simulink model "simulink_scheme_task32"  (R2023b)
settings: Solver=ode4  StartTime=0.0  StopTime=simulationParameters.T_sim  FixedStep=simulationParameters.T_integration  RelTol=1e-3
values from neighbouring files (symbols this model uses):
  nInput = size(B,2)    [buildCondMatrices.m]    (also in main_task31.m; main_task32.m; main_task33.m)
  patientParameters = loadPatientParameter('patient#001')    [main_task32.m]    (also in main_task33.m = loadPatientParameter(patientName))
  predictedHorizon = 100    [main_task31.m]    (also in main_task32.m; main_task33.m)
  predictionData = buildCondMatrices(A,B,C,Q,R,F,f,predictedHorizon)    [main_task31.m]    (also in main_task32.m; main_task33.m)
  simulationParameters = loadSimulationParameter    [main_task31.m]    (also in main_task32.m; main_task33.m)
undefined symbols (not defined in the file or in its folder): MPCcontroller
settings Model: Creator=william  LastModifiedBy=william
settings DataIOCC: ReturnWorkspaceOutputs=off
settings ConfigComp: CovBoundaryAbsTol=1.0e-5

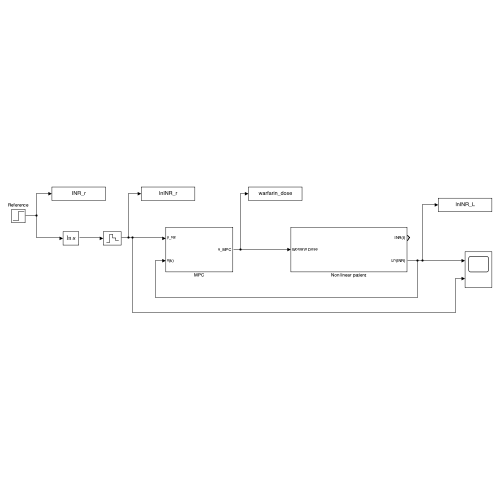
[thumbnail: Simulink's stored preview of the top-level diagram]
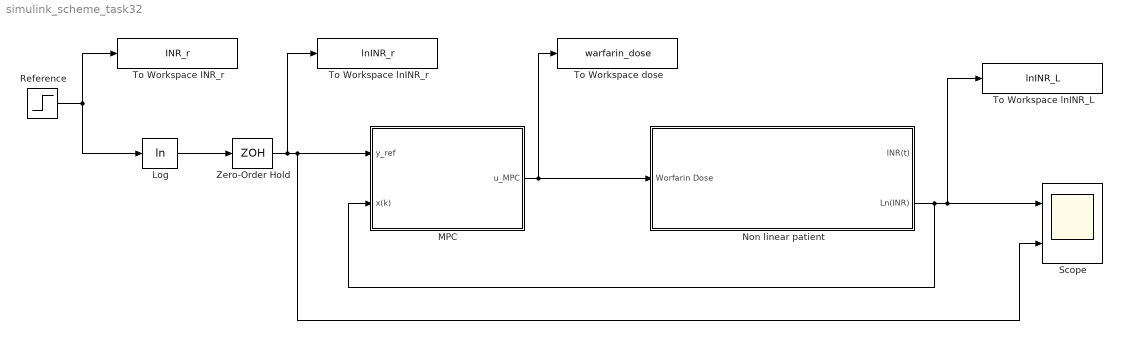
== system simulink_scheme_task32 ==
  Log : Math  Operator=log
  MPC : Subsystem
  Non linear patient : Subsystem
  Reference : Step  Time=2*24  Before=1  After=2.5  SampleTime=simulationParameters.Ts
  Scope : Scope  NumInputPorts=2
  To Workspace INR_r : ToWorkspace  VariableName=INR_r  SaveFormat=Structure With Time  SampleTime=-1
  To Workspace dose : ToWorkspace  VariableName=warfarin_dose  SaveFormat=Structure With Time  SampleTime=-1
  To Workspace lnINR_L : ToWorkspace  VariableName=lnINR_L  SaveFormat=Structure With Time  SampleTime=-1
  To Workspace lnINR_r : ToWorkspace  VariableName=lnINR_r  SaveFormat=Structure With Time  SampleTime=-1
  Zero-Order Hold : ZeroOrderHold  SampleTime=simulationParameters.Ts
  wires:
  Reference/1 -> Log/1, To Workspace INR_r/1
  Log/1 -> Zero-Order Hold/1
  Zero-Order Hold/1 -> Scope/2, MPC/1(y_ref), To Workspace lnINR_r/1
  MPC/1(u_MPC) -> Non linear patient/1(Worfarin Dose), To Workspace dose/1
  Non linear patient/2(Ln(INR)) -> To Workspace lnINR_L/1, Scope/1, MPC/2(x(k))

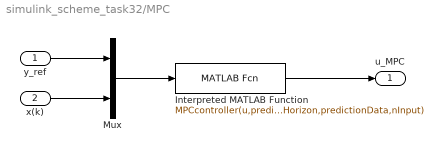
== system simulink_scheme_task32/MPC ==
  y_ref : Inport
  x(k) : Inport  Port=2
  Interpreted MATLAB Function : MATLABFcn  MATLABFcn=MPCcontroller(u,predictedHorizon,predictionData,nInput)
  Mux : Mux  Inputs=2
  u_MPC : Outport
  wires:
  y_ref/1 -> Mux/1
  x(k)/1 -> Mux/2
  Mux/1 -> Interpreted MATLAB Function/1
  Interpreted MATLAB Function/1 -> u_MPC/1

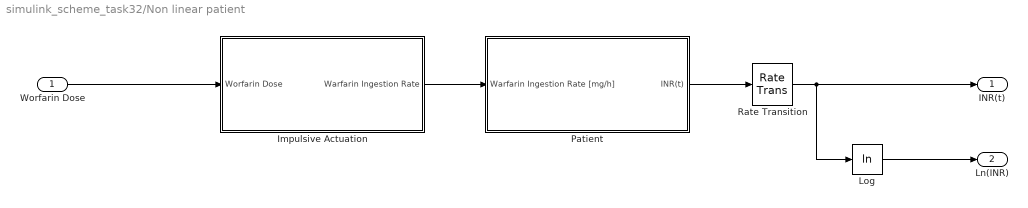
== system simulink_scheme_task32/Non linear patient ==
  Worfarin Dose : Inport
  Impulsive Actuation : Subsystem
  Log : Math  Operator=log
  Patient : Subsystem
  Rate Transition : RateTransition  InitialCondition=patientParameters.BASE  OutPortSampleTime=simulationParameters.Ts
  INR(t) : Outport
  Ln(INR) : Outport  Port=2
  wires:
  Rate Transition/1 -> INR(t)/1, Log/1
  Worfarin Dose/1 -> Impulsive Actuation/1(Worfarin Dose)
  Impulsive Actuation/1(Warfarin Ingestion Rate) -> Patient/1("Warfarin Ingestion Rate [mg/h] ")
  Patient/1(INR(t)) -> Rate Transition/1
  Log/1 -> Ln(INR)/1

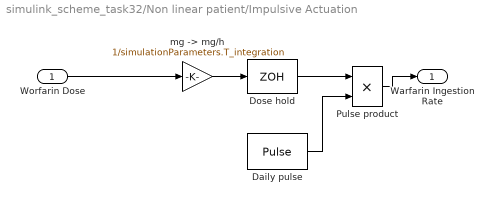
== system simulink_scheme_task32/Non linear patient/Impulsive Actuation ==
  Worfarin Dose : Inport
  Daily pulse : DiscretePulseGenerator  Period=simulationParameters.Ts/simulationParameters.T_integration  SampleTime=simulationParameters.T_integration
  Dose hold : ZeroOrderHold  SampleTime=simulationParameters.T_integration
  Pulse product : Product  Inputs=**
  "mg -> mg/h" : Gain  Gain=1/simulationParameters.T_integration
  Warfarin Ingestion Rate : Outport
  wires:
  Worfarin Dose/1 -> "mg -> mg/h"/1
  "mg -> mg/h"/1 -> Dose hold/1
  Dose hold/1 -> Pulse product/1
  Daily pulse/1 -> Pulse product/2
  Pulse product/1 -> Warfarin Ingestion Rate/1

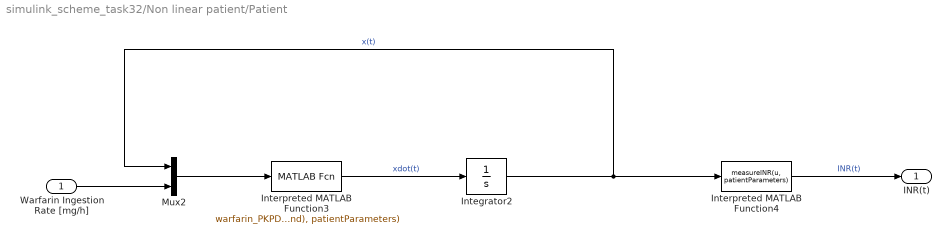
== system simulink_scheme_task32/Non linear patient/Patient ==
  "Warfarin Ingestion Rate [mg/h] " : Inport
  Integrator2 : Integrator  InitialCondition=[patientParameters.x0,patientParameters.appearance.x0]
  Interpreted MATLAB Function3 : MATLABFcn  MATLABFcn=warfarin_PKPD_model(u(1:end-1), u(end), patientParameters)  OutputDimensions=8
  Interpreted MATLAB Function4 : MATLABFcn  MATLABFcn=measureINR(u, patientParameters)
  Mux2 : Mux  Inputs=2
  INR(t) : Outport
  wires:
  Interpreted MATLAB Function3/1 -> Integrator2/1  "xdot(t)"
  Interpreted MATLAB Function4/1 -> INR(t)/1  "INR(t)"
  Integrator2/1 -> Mux2/1, Interpreted MATLAB Function4/1  "x(t)"
  Mux2/1 -> Interpreted MATLAB Function3/1
  "Warfarin Ingestion Rate [mg/h] "/1 -> Mux2/2
